simulink model "s_c107m32k_vlbi"  (R2018a)
settings: Solver=VariableStepDiscrete  StartTime=0.0  StopTime=(2^15)*10  RelTol=1e-3
undefined symbols (not defined in the file): fft_stages, n_bits_xengs
libraries: xbsIndex_r4 x23049, casper_library_misc x45, xps_library x4, casper_library_scopes x3, simulink x2
(part 24 of 201)

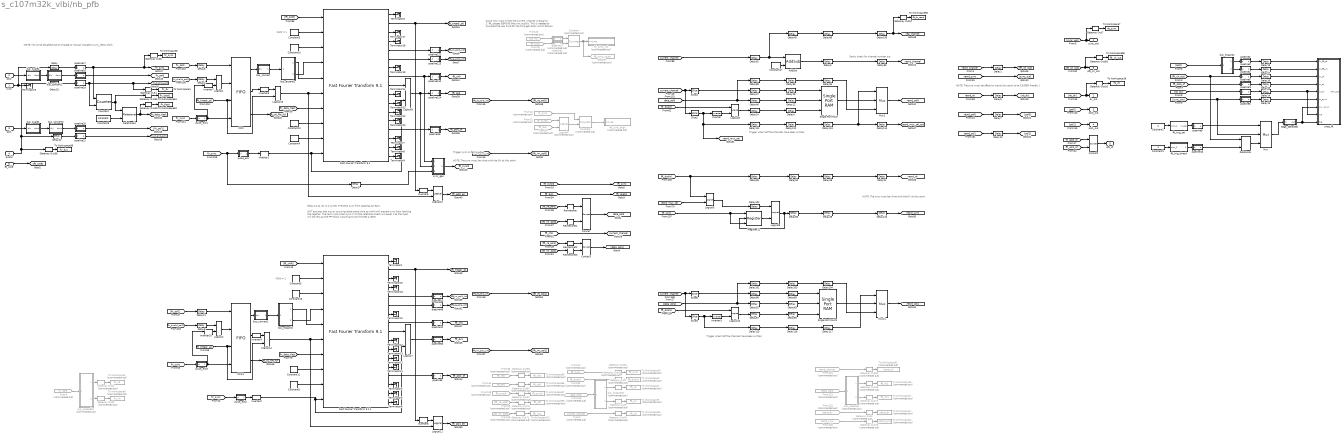
== system s_c107m32k_vlbi/nb_pfb ==
  note: FWD = 1
  note: NOTE: Init script Disabled due to change to manual change to sync_delay block
  note: NOTE: The sync must be inline with the DV at this point
  note: Trigger sync on falling edge
  note: NOT ensures that a sync occuring atthe same time as ch=0 will prevent
      | sync from latching the register. The next cycle when sync in =0 the relational check
      | will equal 1  as the input will be zero as the FFT block would have just finished a reset.
  note: Delay=2 as rst is 2 cycles. Prevents sync from popping out early
  note: Sanity check for channel number out
  note: Trigger when half the channels have been written
  note: Count how many times the current_channel
      | is equal to 2^fft_stages BEFORE the sync occurs.
      | This is needed to compute the new time for the time gen
      | block which follows.
  note: Trigger when half the channels have been written
  note: NOTE: The sync must be inline with the DV at this point
  note: FWD = 1
  note: NOTE: The sync must be offset by one at this point to be CASPER friendly :)
  sync : Inport
  pol0 : Inport  Port=2
  pol1 : Inport  Port=3
  dvalid : Inport  Port=4
  fft_shift : Inport  Port=5
  AddSub : xbsIndex_r4/AddSub  mode=Subtraction  use_carryin=off  use_carryout=off  en=off  latency=1  precision=User Defined  arith_type=Unsigned  n_bits=fft_stages-1  bin_pt=0  quantization=Truncate  overflow=Wrap  use_behavioral_HDL=off  hw_selection=Fabric  pipelined=off  dbl_ovrd=off  block_type=addsub
  Concat : xbsIndex_r4/Concat  num_inputs=2  dbl_ovrd=off  block_type=concat
  Concat2 : xbsIndex_r4/Concat  num_inputs=2  dbl_ovrd=off  block_type=concat
  Concat3 : xbsIndex_r4/Concat  num_inputs=2  dbl_ovrd=off  block_type=concat
  Constant1 : Constant  SampleTime=1
  Constant10 : xbsIndex_r4/Constant  const=1  gui_display_data_type=Boolean  arith_type=Boolean  n_bits=1  bin_pt=0  preci_type=Single  exp_width=8  frac_width=24  explicit_period=on  period=1  equ=P=C  opselect=C  inp2=PCIN>>17  opr=+  inp1=P  carry=CIN  dbl_ovrd=off  block_type=constant
  Constant11 : xbsIndex_r4/Constant  const=1  gui_display_data_type=Boolean  arith_type=Boolean  n_bits=18  bin_pt=17  preci_type=Single  exp_width=8  frac_width=24  explicit_period=on  period=1  equ=P=C  opselect=C  inp2=PCIN>>17  opr=+  inp1=P  carry=CIN  dbl_ovrd=off  block_type=constant
  Constant12 : xbsIndex_r4/Constant  const=1  gui_display_data_type=Boolean  arith_type=Boolean  n_bits=18  bin_pt=17  preci_type=Single  exp_width=8  frac_width=24  explicit_period=on  period=1  equ=P=C  opselect=C  inp2=PCIN>>17  opr=+  inp1=P  carry=CIN  dbl_ovrd=off  block_type=constant
  Constant13 : xbsIndex_r4/Constant  const=1  gui_display_data_type=Boolean  arith_type=Boolean  n_bits=1  bin_pt=0  preci_type=Single  exp_width=8  frac_width=24  explicit_period=on  period=1  equ=P=C  opselect=C  inp2=PCIN>>17  opr=+  inp1=P  carry=CIN  dbl_ovrd=off  block_type=constant
  Constant17 : xbsIndex_r4/Constant  const=2^(fft_stages-2)  gui_display_data_type=Fixed-point  arith_type=Unsigned  n_bits=fft_stages-1  bin_pt=0  preci_type=Single  exp_width=8  frac_width=24  explicit_period=on  period=1  equ=P=C  opselect=C  inp2=PCIN>>17  opr=+  inp1=P  carry=CIN  dbl_ovrd=off  block_type=constant
  Constant2 : Constant  SampleTime=1
  Constant3 : xbsIndex_r4/Constant  const=1  gui_display_data_type=Fixed-point  arith_type=Unsigned  n_bits=1  bin_pt=0  preci_type=Single  exp_width=8  frac_width=24  explicit_period=on  period=1  equ=P=C  opselect=C  inp2=PCIN>>17  opr=+  inp1=P  carry=CIN  dbl_ovrd=off  block_type=constant
  Constant4 : xbsIndex_r4/Constant  const=1.0  gui_display_data_type=Boolean  arith_type=Boolean  n_bits=16  bin_pt=14  preci_type=Single  exp_width=8  frac_width=24  explicit_period=on  period=1  equ=P=C  opselect=C  inp2=PCIN>>17  opr=+  inp1=P  carry=CIN  dbl_ovrd=off  block_type=constant
  Constant5 : xbsIndex_r4/Constant  const=1  gui_display_data_type=Fixed-point  arith_type=Unsigned  n_bits=1  bin_pt=0  preci_type=Single  exp_width=8  frac_width=24  explicit_period=on  period=1  equ=P=C  opselect=C  inp2=PCIN>>17  opr=+  inp1=P  carry=CIN  dbl_ovrd=off  block_type=constant
  Constant8 : xbsIndex_r4/Constant  const=1  gui_display_data_type=Boolean  arith_type=Boolean  n_bits=18  bin_pt=17  preci_type=Single  exp_width=8  frac_width=24  explicit_period=on  period=1  equ=P=C  opselect=C  inp2=PCIN>>17  opr=+  inp1=P  carry=CIN  dbl_ovrd=off  block_type=constant
  Constant9 : xbsIndex_r4/Constant  const=(2^(fft_stages-1))-1  gui_display_data_type=Fixed-point  arith_type=Unsigned  n_bits=fft_stages+1  bin_pt=0  preci_type=Single  exp_width=8  frac_width=24  explicit_period=on  period=1  equ=P=C  opselect=C  inp2=PCIN>>17  opr=+  inp1=P  carry=CIN  dbl_ovrd=off  block_type=constant
  Counter3 : xbsIndex_r4/Counter  cnt_type=Free Running  cnt_to=Inf  operation=Up  start_count=0  cnt_by_val=1  arith_type=Unsigned  n_bits=fft_stages-1  bin_pt=0  load_pin=off  rst=on  en=on  explicit_period=on  period=1  use_behavioral_HDL=off  implementation=Fabric  dbl_ovrd=off  block_type=counter
  Counter4 : xbsIndex_r4/Counter  Commented=on  cnt_type=Free Running  cnt_to=Inf  operation=Up  start_count=0  cnt_by_val=1  arith_type=Unsigned  n_bits=11  bin_pt=0  load_pin=off  rst=on  en=on  explicit_period=on  period=1  use_behavioral_HDL=off  implementation=DSP48  dbl_ovrd=off  block_type=counter
      settings: block_version=11.4
  Counter5 : xbsIndex_r4/Counter  Commented=on  cnt_type=Free Running  cnt_to=Inf  operation=Up  start_count=0  cnt_by_val=1  arith_type=Unsigned  n_bits=11  bin_pt=0  load_pin=off  rst=on  en=on  explicit_period=on  period=1  use_behavioral_HDL=off  implementation=DSP48  dbl_ovrd=off  block_type=counter
      settings: block_version=11.4
  Delay{,1,3..5,7,10,12..22,24,45..50,55,63,65,86..88,90..96,99..104,110..117} (52 alike) : xbsIndex_r4/Delay  rst=off  infoeditControl=Selection of Reset will increase slice count due to use of real FFs and instead of SRLs  en=off  latency=1  reg_retiming=off  dbl_ovrd=off  block_type=delay
      Delay1 settings: infoedit=Hardware notes: A delay line is a chain, each link of which is an SRL16 or SRL32 followed by a flip-flop.
      Delay10 settings: infoedit=Hardware notes: A delay line is a chain, each link of which is an SRL16 or SRL32 followed by a flip-flop.
      Delay100 settings: infoedit=Hardware notes: A delay line is a chain, each link of which is an SRL16 or SRL32 followed by a flip-flop.
      Delay101 settings: infoedit=Hardware notes: A delay line is a chain, each link of which is an SRL16 or SRL32 followed by a flip-flop.
      Delay102 settings: infoedit=Hardware notes: A delay line is a chain, each link of which is an SRL16 or SRL32 followed by a flip-flop.
      Delay103 settings: infoedit=Hardware notes: A delay line is a chain, each link of which is an SRL16 or SRL32 followed by a flip-flop.
      Delay104 settings: infoedit=Hardware notes: A delay line is a chain, each link of which is an SRL16 or SRL32 followed by a flip-flop.
      Delay110 settings: infoedit=Hardware notes: A delay line is a chain, each link of which is an SRL16 or SRL32 followed by a flip-flop.
      Delay111 settings: infoedit=Hardware notes: A delay line is a chain, each link of which is an SRL16 or SRL32 followed by a flip-flop.
      Delay112 settings: infoedit=Hardware notes: A delay line is a chain, each link of which is an SRL16 or SRL32 followed by a flip-flop.
      Delay113 settings: infoedit=Hardware notes: A delay line is a chain, each link of which is an SRL16 or SRL32 followed by a flip-flop.
      Delay114 settings: infoedit=Hardware notes: A delay line is a chain, each link of which is an SRL16 or SRL32 followed by a flip-flop.
      Delay115 settings: infoedit=Hardware notes: A delay line is a chain, each link of which is an SRL16 or SRL32 followed by a flip-flop.
      Delay116 settings: infoedit=Hardware notes: A delay line is a chain, each link of which is an SRL16 or SRL32 followed by a flip-flop.
      Delay117 settings: infoedit=Hardware notes: A delay line is a chain, each link of which is an SRL16 or SRL32 followed by a flip-flop.
      Delay12 settings: infoedit=Hardware notes: A delay line is a chain, each link of which is an SRL16 or SRL32 followed by a flip-flop.
      Delay13 settings: infoedit=Hardware notes: A delay line is a chain, each link of which is an SRL16 or SRL32 followed by a flip-flop.
      Delay14 settings: infoedit=Hardware notes: A delay line is a chain, each link of which is an SRL16 or SRL32 followed by a flip-flop.
      Delay15 settings: infoedit=Hardware notes: A delay line is a chain, each link of which is an SRL16 or SRL32 followed by a flip-flop.
      Delay16 settings: infoedit=Hardware notes: A delay line is a chain, each link of which is an SRL16 or SRL32 followed by a flip-flop.
      Delay17 settings: infoedit=Hardware notes: A delay line is a chain, each link of which is an SRL16 or SRL32 followed by a flip-flop.
      Delay18 settings: infoedit=Hardware notes: A delay line is a chain, each link of which is an SRL16 or SRL32 followed by a flip-flop.
      Delay19 settings: infoedit=Hardware notes: A delay line is a chain, each link of which is an SRL16 or SRL32 followed by a flip-flop.
      Delay21 settings: infoedit=Hardware notes: A delay line is a chain, each link of which is an SRL16 or SRL32 followed by a flip-flop.
      Delay24 settings: infoedit=Hardware notes: A delay line is a chain, each link of which is an SRL16 or SRL32 followed by a flip-flop.
      Delay3 settings: infoedit=Hardware notes: A delay line is a chain, each link of which is an SRL16 or SRL32 followed by a flip-flop.
      Delay4 settings: infoedit=Hardware notes: A delay line is a chain, each link of which is an SRL16 or SRL32 followed by a flip-flop.
      Delay45 settings: infoedit=Hardware notes: A delay line is a chain, each link of which is an SRL16 or SRL32 followed by a flip-flop.
      Delay46 settings: infoedit=Hardware notes: A delay line is a chain, each link of which is an SRL16 or SRL32 followed by a flip-flop.
      Delay47 settings: infoedit=Hardware notes: A delay line is a chain, each link of which is an SRL16 or SRL32 followed by a flip-flop.
      Delay48 settings: infoedit=Hardware notes: A delay line is a chain, each link of which is an SRL16 or SRL32 followed by a flip-flop.
      Delay49 settings: infoedit=Hardware notes: A delay line is a chain, each link of which is an SRL16 or SRL32 followed by a flip-flop.
      Delay5 settings: infoedit=Hardware notes: A delay line is a chain, each link of which is an SRL16 or SRL32 followed by a flip-flop.
      Delay50 settings: infoedit=Hardware notes: A delay line is a chain, each link of which is an SRL16 or SRL32 followed by a flip-flop.
      Delay55 settings: infoedit=Hardware notes: A delay line is a chain, each link of which is an SRL16 or SRL32 followed by a flip-flop.
      Delay63 settings: infoedit=Hardware notes: A delay line is a chain, each link of which is an SRL16 or SRL32 followed by a flip-flop.
      Delay65 settings: infoedit=Hardware notes: A delay line is a chain, each link of which is an SRL16 or SRL32 followed by a flip-flop.
      Delay7 settings: infoedit=Hardware notes: A delay line is a chain, each link of which is an SRL16 or SRL32 followed by a flip-flop.
      Delay86 settings: infoedit=Hardware notes: A delay line is a chain, each link of which is an SRL16 or SRL32 followed by a flip-flop.
      Delay87 settings: infoedit=Hardware notes: A delay line is a chain, each link of which is an SRL16 or SRL32 followed by a flip-flop.
      Delay88 settings: infoedit=Hardware notes: A delay line is a chain, each link of which is an SRL16 or SRL32 followed by a flip-flop.
      Delay90 settings: infoedit=Hardware notes: A delay line is a chain, each link of which is an SRL16 or SRL32 followed by a flip-flop.
      Delay91 settings: infoedit=Hardware notes: A delay line is a chain, each link of which is an SRL16 or SRL32 followed by a flip-flop.
      Delay92 settings: infoedit=Hardware notes: A delay line is a chain, each link of which is an SRL16 or SRL32 followed by a flip-flop.
      Delay93 settings: infoedit=Hardware notes: A delay line is a chain, each link of which is an SRL16 or SRL32 followed by a flip-flop.
      Delay94 settings: infoedit=Hardware notes: A delay line is a chain, each link of which is an SRL16 or SRL32 followed by a flip-flop.
      Delay95 settings: infoedit=Hardware notes: A delay line is a chain, each link of which is an SRL16 or SRL32 followed by a flip-flop.
      Delay96 settings: infoedit=Hardware notes: A delay line is a chain, each link of which is an SRL16 or SRL32 followed by a flip-flop.
      Delay99 settings: infoedit=Hardware notes: A delay line is a chain, each link of which is an SRL16 or SRL32 followed by a flip-flop.
  Delay{2,6,8,11} (4 alike) : xbsIndex_r4/Delay  rst=off  infoeditControl=Selection of Reset will increase slice count due to use of real FFs and instead of SRLs  en=off  latency=10  reg_retiming=off  dbl_ovrd=off  block_type=delay
      settings: infoedit=Hardware notes: A delay line is a chain, each link of which is an SRL16 or SRL32 followed by a flip-flop.
  Delay9 : xbsIndex_r4/Delay  rst=off  infoeditControl=Selection of Reset will increase slice count due to use of real FFs and instead of SRLs  en=off  latency=2  reg_retiming=off  dbl_ovrd=off  block_type=delay
      settings: infoedit=Hardware notes: A delay line is a chain, each link of which is an SRL16 or SRL32 followed by a flip-flop.
  FIFO : xbsIndex_r4/FIFO  mem_type=Distributed RAM  performance_options=First_Word_Fall_Through  embedded_registers=off  depth=16  percent_nbits=1  rst=on  rst_latency=1  en=off  use_dcount=off  use_percent_full_port=off  use_almost_empty=off  almost_empty_thresh=2  use_almost_full=off  use_rd_rst_busy=off  use_wr_rst_busy=off  almost_full_thresh=14  explicit_period=off  dbl_ovrd=off  block_type=fifo
  FIFO1 : xbsIndex_r4/FIFO  mem_type=Distributed RAM  performance_options=First_Word_Fall_Through  embedded_registers=off  depth=16  percent_nbits=1  rst=on  rst_latency=1  en=off  use_dcount=off  use_percent_full_port=off  use_almost_empty=off  almost_empty_thresh=2  use_almost_full=off  use_rd_rst_busy=off  use_wr_rst_busy=off  almost_full_thresh=14  explicit_period=off  dbl_ovrd=off  block_type=fifo
  "Fast Fourier Transform 9.1 " : xbsIndex_r4/Fast Fourier Transform 9.1   transform_length=32768  target_clock_frequency=240  target_data_throughput=50  implementation_options=pipelined_streaming_io  run_time_configurable_transform_length=off  phase_factor_width=18  scaling_options=scaled  rounding_modes=convergent_rounding  aclken=off  aresetn=on  output_ordering=natural_order  cyclic_prefix_insertion=off  throttle_scheme=nonrealtime  xk_index=on  ovflo=on  trim_axipin_name=on  memory_options_data=block_ram  memory_options_phase_factors=block_ram  number_of_stages_using_block_ram_for_data_and_phase_factors=6  memory_options_reorder=block_ram  memory_options_hybrid=off  complex_mult_type=use_mults_performance  butterfly_type=use_xtremedsp_slices  simulation_type=hybrid_sim  simulation_model=sysgen:xfftv9_cmodel  data_path_portlist={ 's_axis_data_tdata', 'm_axis_data_tdata', 'm_axis_status_tdata', 'event_fft_overflow' }  channels=1  input_ordering=natural_order  input_width=16  ip_name=Fast Fourier Transform  ip_version=9.1  dsptool_ready=true  ipcore_usecache=true  ipcore_useipmodelcache=true  wrapper_available=true  port_translation_map={ 'aclken' => 'en', 'aresetn' => 'rst'}  data_format=fixed_point  block_type=xfft_v9_1
  Fast Fourier Transform 9.1 1 : xbsIndex_r4/Fast Fourier Transform 9.1   transform_length=32768  target_clock_frequency=240  target_data_throughput=50  implementation_options=pipelined_streaming_io  run_time_configurable_transform_length=off  phase_factor_width=18  scaling_options=scaled  rounding_modes=convergent_rounding  aclken=off  aresetn=on  output_ordering=natural_order  cyclic_prefix_insertion=off  throttle_scheme=nonrealtime  xk_index=on  ovflo=on  trim_axipin_name=on  memory_options_data=block_ram  memory_options_phase_factors=block_ram  number_of_stages_using_block_ram_for_data_and_phase_factors=6  memory_options_reorder=block_ram  memory_options_hybrid=off  complex_mult_type=use_mults_performance  butterfly_type=use_xtremedsp_slices  simulation_type=hybrid_sim  simulation_model=sysgen:xfftv9_cmodel  data_path_portlist={ 's_axis_data_tdata', 'm_axis_data_tdata', 'm_axis_status_tdata', 'event_fft_overflow' }  channels=1  input_ordering=natural_order  input_width=16  ip_name=Fast Fourier Transform  ip_version=9.1  dsptool_ready=true  ipcore_usecache=true  ipcore_useipmodelcache=true  wrapper_available=true  port_translation_map={ 'aclken' => 'en', 'aresetn' => 'rst'}  data_format=fixed_point  block_type=xfft_v9_1
  From108 : From  Commented=on  GotoTag=fft_sync0  TagVisibility=global
  From123 : From  Commented=on  GotoTag=reord_pol0  TagVisibility=global
  From124 : From  Commented=on  GotoTag=reord_channel  TagVisibility=global
  From125 : From  Commented=on  GotoTag=reord_dv  TagVisibility=global
  From126 : From  Commented=on  GotoTag=reord_sync  TagVisibility=global
  From140 : From  Commented=on  GotoTag=data_pol0  TagVisibility=global
  From2 : From  Commented=on  GotoTag=current_channel  TagVisibility=global
  From20 : From  Commented=on  GotoTag=fft_sync  TagVisibility=global
  From26 : From  Commented=on  GotoTag=cnt_rst  TagVisibility=global
      settings: CloseFcn=tagdialog Close
  From28 : From  Commented=on  GotoTag=fft_re_pol0
  From30 : From  Commented=on  GotoTag=fft_dvalid  TagVisibility=global
  From31 : From  Commented=on  GotoTag=fft_sync0  TagVisibility=global
  From32 : From  Commented=on  GotoTag=fft_sync  TagVisibility=global
  From33 : From  Commented=on  GotoTag=fft_im_pol0
  From34 : From  Commented=on  GotoTag=fft_dv0  TagVisibility=global
  From38 : From  Commented=on  GotoTag=fft_ch0  TagVisibility=global
  From4 : From  Commented=on  GotoTag=fir_pol0  TagVisibility=global
  From40 : From  Commented=on  GotoTag=fft_dv0  TagVisibility=global
  From42 : From  Commented=on  GotoTag=fir_sync  TagVisibility=global
  Gateway Out{1,6..7,18,36,48,53,57,83} (9 alike) : xbsIndex_r4/Gateway Out  inherit_from_input=off  hdl_port=on  rows=1  columns=1  UseAsDAC=off  DACChannel='1'  interface=None  automatic_assignment=on  address_offset=hex2dec('00')  intf_name=''  intf_description=''  timing_constraint=None  locs_specified=off  LOCs={}  io_standard={}  block_type=gatewayout
  Gateway Out{2..5,8,15..17,34,37,50..52,66..67,70..71} (17 alike) : xbsIndex_r4/Gateway Out  Commented=on  inherit_from_input=off  hdl_port=on  rows=1  columns=1  UseAsDAC=off  DACChannel='1'  interface=None  automatic_assignment=on  address_offset=hex2dec('00')  intf_name=''  intf_description=''  timing_constraint=None  locs_specified=off  LOCs={}  io_standard={}  block_type=gatewayout
  Goto29 : Goto  Commented=on  GotoTag=fft_sync_count  TagVisibility=global
  Inverter{,1..3,5..10} (10 alike) : xbsIndex_r4/Inverter  en=off  latency=0  dbl_ovrd=off  block_type=inv
  Logical{1..2,5..14} (12 alike) : xbsIndex_r4/Logical  logical_function=AND  inputs=2  en=off  latency=0  precision=Full  arith_type=Unsigned  n_bits=16  bin_pt=0  align_bp=on  dbl_ovrd=off  block_type=logical
  Logical4 : xbsIndex_r4/Logical  Commented=on  logical_function=AND  inputs=2  en=off  latency=0  precision=Full  arith_type=Unsigned  n_bits=16  bin_pt=0  align_bp=on  dbl_ovrd=off  block_type=logical
  Mux : xbsIndex_r4/Mux  inputs=2  en=off  latency=1  precision=Full  arith_type=Unsigned  n_bits=16  bin_pt=14  quantization=Truncate  overflow=Wrap  dbl_ovrd=off  block_type=mux
  Mux1 : xbsIndex_r4/Mux  inputs=2  en=off  latency=1  precision=Full  arith_type=Unsigned  n_bits=16  bin_pt=14  quantization=Truncate  overflow=Wrap  dbl_ovrd=off  block_type=mux
  Mux11 : xbsIndex_r4/Mux  inputs=2  en=off  latency=1  precision=Full  arith_type=Unsigned  n_bits=16  bin_pt=14  quantization=Truncate  overflow=Wrap  dbl_ovrd=off  block_type=mux
  Register12 : xbsIndex_r4/Register  init=0  rst=on  en=on  dbl_ovrd=off  block_type=register
  Reinterpret{,1..3} (4 alike) : xbsIndex_r4/Reinterpret  force_arith_type=on  arith_type=Unsigned  force_bin_pt=on  bin_pt=0  block_type=reinterpret
  Relational : xbsIndex_r4/Relational  mode=a=b  op_type=Bool  en=off  latency=2  dbl_ovrd=off  block_type=relational
  Relational4 : xbsIndex_r4/Relational  mode=a=b  op_type=Bool  en=off  latency=1  dbl_ovrd=off  block_type=relational
  Single Port RAM : xbsIndex_r4/Single Port RAM  depth=2^(fft_stages-2)  initVector=0  distributed_mem=Block RAM  write_mode=Read Before Write  rst=off  init_reg=0  en=off  latency=1  optimize=Area  dbl_ovrd=off  block_type=spram
  Single Port RAM1 : xbsIndex_r4/Single Port RAM  depth=2^(fft_stages-2)  initVector=0  distributed_mem=Block RAM  write_mode=Read Before Write  rst=off  init_reg=0  en=off  latency=1  optimize=Area  dbl_ovrd=off  block_type=spram
  Slice2 : xbsIndex_r4/Slice  nbits=1  boolean_output=on  mode=Lower Bit Location + Width  bit1=0  base1=MSB of Input  bit0=fft_stages-2  base0=LSB of Input  dbl_ovrd=off  block_type=slice
  Slice3 : xbsIndex_r4/Slice  nbits=1  boolean_output=on  mode=Lower Bit Location + Width  bit1=0  base1=MSB of Input  bit0=fft_stages-2  base0=LSB of Input  dbl_ovrd=off  block_type=slice
  Slice4 : xbsIndex_r4/Slice  nbits=fft_stages-2  boolean_output=off  mode=Lower Bit Location + Width  bit1=0  base1=MSB of Input  bit0=0  base0=LSB of Input  dbl_ovrd=off  block_type=slice
  Slice6 : xbsIndex_r4/Slice  nbits=fft_stages-2  boolean_output=off  mode=Lower Bit Location + Width  bit1=0  base1=MSB of Input  bit0=0  base0=LSB of Input  dbl_ovrd=off  block_type=slice
  Terminator{1..13,15..24} (23 alike) : Terminator
  To Workspace1 : ToWorkspace  VariableName=fir_dv  SaveFormat=Timeseries  SampleTime=-1
  To Workspace15 : ToWorkspace  Commented=on  VariableName=fft_re1  SaveFormat=Timeseries  SampleTime=-1
  To Workspace16 : ToWorkspace  Commented=on  VariableName=fft_sync  SaveFormat=Timeseries  SampleTime=-1
  To Workspace17 : ToWorkspace  Commented=on  VariableName=fft_im1  SaveFormat=Timeseries  SampleTime=-1
  To Workspace19 : ToWorkspace  VariableName=nb_dv  SaveFormat=Timeseries  SampleTime=-1
  To Workspace2 : ToWorkspace  Commented=on  VariableName=fft_re  SaveFormat=Timeseries  SampleTime=-1
  To Workspace3 : ToWorkspace  Commented=on  VariableName=fft_dvalid  SaveFormat=Timeseries  SampleTime=-1
  To Workspace32 : ToWorkspace  Commented=on  VariableName=fft_ch  SaveFormat=Timeseries  SampleTime=-1
  To Workspace36 : ToWorkspace  VariableName=fir_dv1  SaveFormat=Timeseries  SampleTime=-1
  To Workspace37 : ToWorkspace  Commented=on  VariableName=fft_sync0  SaveFormat=Timeseries  SampleTime=-1
  To Workspace4 : ToWorkspace  Commented=on  VariableName=fir_re  SaveFormat=Timeseries  SampleTime=-1
  To Workspace42 : ToWorkspace  Commented=on  VariableName=reord_sync  SaveFormat=Timeseries  SampleTime=-1
  To Workspace47 : ToWorkspace  Commented=on  VariableName=reord_dv  SaveFormat=Timeseries  SampleTime=-1
  To Workspace5 : ToWorkspace  Commented=on  VariableName=fft_im  SaveFormat=Timeseries  SampleTime=-1
  To Workspace51 : ToWorkspace  Commented=on  VariableName=reord_ch  SaveFormat=Timeseries  SampleTime=-1
  To Workspace53 : ToWorkspace  VariableName=fir_tlast  SaveFormat=Timeseries  SampleTime=-1
  To Workspace54 : ToWorkspace  VariableName=fir_tlast1  SaveFormat=Timeseries  SampleTime=-1
  To Workspace58 : ToWorkspace  VariableName=fft_ch_reord  SaveFormat=Timeseries  SampleTime=-1
  To Workspace6 : ToWorkspace  VariableName=fir_sync  SaveFormat=Timeseries  SampleTime=-1
  To Workspace65 : ToWorkspace  Commented=on  VariableName=fft_ch0  SaveFormat=Timeseries  SampleTime=-1
  To Workspace66 : ToWorkspace  Commented=on  VariableName=fft_dv0  SaveFormat=Timeseries  SampleTime=-1
  To Workspace69 : ToWorkspace  Commented=on  VariableName=fft_re2  SaveFormat=Timeseries  SampleTime=-1
  To Workspace7 : ToWorkspace  VariableName=nb_sync  SaveFormat=Timeseries  SampleTime=-1
  To Workspace70 : ToWorkspace  Commented=on  VariableName=fft_im2  SaveFormat=Timeseries  SampleTime=-1
  To Workspace8 : ToWorkspace  Commented=on  VariableName=fir_im  SaveFormat=Timeseries  SampleTime=-1
  To Workspace85 : ToWorkspace  VariableName=fft_ch_out  SaveFormat=Timeseries  SampleTime=-1
  bus_convert : Subsystem  AncestorBlock=casper_library_bus/bus_convert  mask(bus_convert){n_bits_in=[18 18], bin_pt_in=[17 17], cmplx=off, n_bits_out=[22 22], bin_pt_out=[21 21], quantization=0, overflow=0, csp_latency=0, of=off, misc=off}
      mask prompts: n_bits_in "input bit widths"; bin_pt_in "input binary points"; cmplx "input complex"; n_bits_out "output bit widths"; bin_pt_out "output binary points"; quantization "quantization strategy (Truncate=0, Round  (unbiased: +/- Inf)=1, Round (unbiased: Even Values)=2)"; overflow "overflow strategy (Wrap=0, Saturate=1, Flag as error=2)"; csp_latency "latency"; of "overflow indication"; misc "misc support"
      mask help: Convert components of busses
      mask init: same as s_c107m32k_vlbi/DDC/bus_convert
  bus_convert1 : Subsystem  AncestorBlock=casper_library_bus/bus_convert  mask(bus_convert){n_bits_in=[18 18], bin_pt_in=[17 17], cmplx=off, n_bits_out=[22 22], bin_pt_out=[21 21], quantization=0, overflow=0, csp_latency=0, of=off, misc=off}
      mask prompts: n_bits_in "input bit widths"; bin_pt_in "input binary points"; cmplx "input complex"; n_bits_out "output bit widths"; bin_pt_out "output binary points"; quantization "quantization strategy (Truncate=0, Round  (unbiased: +/- Inf)=1, Round (unbiased: Even Values)=2)"; overflow "overflow strategy (Wrap=0, Saturate=1, Flag as error=2)"; csp_latency "latency"; of "overflow indication"; misc "misc support"
      mask help: Convert components of busses
      mask init: same as s_c107m32k_vlbi/DDC/bus_convert
  bus_convert2 : Subsystem  AncestorBlock=casper_library_bus/bus_convert  mask(bus_convert){n_bits_in=[18], bin_pt_in=18, cmplx=on, n_bits_out=18, bin_pt_out=17, quantization=2, overflow=1, csp_latency=1, of=off, misc=off}
      mask prompts: n_bits_in "input bit widths"; bin_pt_in "input binary points"; cmplx "input complex"; n_bits_out "output bit widths"; bin_pt_out "output binary points"; quantization "quantization strategy (Truncate=0, Round  (unbiased: +/- Inf)=1, Round (unbiased: Even Values)=2)"; overflow "overflow strategy (Wrap=0, Saturate=1, Flag as error=2)"; csp_latency "latency"; of "overflow indication"; misc "misc support"
      mask help: Convert components of busses
      mask init: same as s_c107m32k_vlbi/DDC/bus_convert
  bus_convert3 : Subsystem  AncestorBlock=casper_library_bus/bus_convert  mask(bus_convert){n_bits_in=[18], bin_pt_in=18, cmplx=on, n_bits_out=18, bin_pt_out=17, quantization=2, overflow=1, csp_latency=1, of=off, misc=off}
      mask prompts: n_bits_in "input bit widths"; bin_pt_in "input binary points"; cmplx "input complex"; n_bits_out "output bit widths"; bin_pt_out "output binary points"; quantization "quantization strategy (Truncate=0, Round  (unbiased: +/- Inf)=1, Round (unbiased: Even Values)=2)"; overflow "overflow strategy (Wrap=0, Saturate=1, Flag as error=2)"; csp_latency "latency"; of "overflow indication"; misc "misc support"
      mask help: Convert components of busses
      mask init: same as s_c107m32k_vlbi/DDC/bus_convert
  bus_expand1 : Subsystem  mask(bus_expand){mode=divisions of equal size, outputNum=2, outputWidth=22, outputBinaryPt=21, outputArithmeticType=1, show_format=off, outputToWorkspace=off, variablePrefix=out, outputToModelAsWell=on}
      mask prompts: outputNum "Number of outputs:"; outputWidth "Output width:"; outputBinaryPt "Output binary point position:"; outputArithmeticType "Output arithmetic type (ufix=0, fix=1, bool=2):"; show_format "Print format string?"; outputToWorkspace "Output to workspace?"; variablePrefix "Variable name prefix:"; outputToModelAsWell "Output to model as well?"
      mask help:
      | Expands a 'bus' made using a bus_create or Xilinx
      | concat block.
      | The input will be divided into the specified number
      | of outputs with the specified arithmetic types.
      | Divisions are made from most significant bit.
      mask init: same as s_c107m32k_vlbi/bus_expand1
      settings: AttributesFormatString=2 outputs
      mask TypeOptions mode: divisions of equal size | divisions of arbitrary size
      mask Callback mode: bus_expand_callback();
      mask Callback outputWidth: bus_expand_callback();
      mask Callback outputToWorkspace: bus_expand_callback();
  bus_expand13 : Subsystem  Commented=on  mask(bus_expand){mode=divisions of equal size, outputNum=2, outputWidth=18, outputBinaryPt=17, outputArithmeticType=1, show_format=off, outputToWorkspace=off, variablePrefix=out, outputToModelAsWell=on}
      mask prompts: outputNum "Number of outputs:"; outputWidth "Output width:"; outputBinaryPt "Output binary point position:"; outputArithmeticType "Output arithmetic type (ufix=0, fix=1, bool=2):"; show_format "Print format string?"; outputToWorkspace "Output to workspace?"; variablePrefix "Variable name prefix:"; outputToModelAsWell "Output to model as well?"
      mask help:
      | Expands a 'bus' made using a bus_create or Xilinx
      | concat block.
      | The input will be divided into the specified number
      | of outputs with the specified arithmetic types.
      | Divisions are made from most significant bit.
      mask init: same as s_c107m32k_vlbi/bus_expand1
      settings: AttributesFormatString=2 outputs
      mask TypeOptions mode: divisions of equal size | divisions of arbitrary size
      mask Callback mode: bus_expand_callback();
      mask Callback outputWidth: bus_expand_callback();
      mask Callback outputToWorkspace: bus_expand_callback();
  bus_expand16 : Subsystem  Commented=on  mask(bus_expand){mode=divisions of equal size, outputNum=2, outputWidth=18, outputBinaryPt=17, outputArithmeticType=1, show_format=off, outputToWorkspace=off, variablePrefix=out, outputToModelAsWell=on}
      mask prompts: outputNum "Number of outputs:"; outputWidth "Output width:"; outputBinaryPt "Output binary point position:"; outputArithmeticType "Output arithmetic type (ufix=0, fix=1, bool=2):"; show_format "Print format string?"; outputToWorkspace "Output to workspace?"; variablePrefix "Variable name prefix:"; outputToModelAsWell "Output to model as well?"
      mask help:
      | Expands a 'bus' made using a bus_create or Xilinx
      | concat block.
      | The input will be divided into the specified number
      | of outputs with the specified arithmetic types.
      | Divisions are made from most significant bit.
      mask init: same as s_c107m32k_vlbi/bus_expand1
      settings: AttributesFormatString=2 outputs
      mask TypeOptions mode: divisions of equal size | divisions of arbitrary size
      mask Callback mode: bus_expand_callback();
      mask Callback outputWidth: bus_expand_callback();
      mask Callback outputToWorkspace: bus_expand_callback();
  bus_expand2 : Subsystem  mask(bus_expand){mode=divisions of equal size, outputNum=2, outputWidth=22, outputBinaryPt=21, outputArithmeticType=1, show_format=off, outputToWorkspace=off, variablePrefix=out, outputToModelAsWell=on}
      mask prompts: outputNum "Number of outputs:"; outputWidth "Output width:"; outputBinaryPt "Output binary point position:"; outputArithmeticType "Output arithmetic type (ufix=0, fix=1, bool=2):"; show_format "Print format string?"; outputToWorkspace "Output to workspace?"; variablePrefix "Variable name prefix:"; outputToModelAsWell "Output to model as well?"
      mask help:
      | Expands a 'bus' made using a bus_create or Xilinx
      | concat block.
      | The input will be divided into the specified number
      | of outputs with the specified arithmetic types.
      | Divisions are made from most significant bit.
      mask init: same as s_c107m32k_vlbi/bus_expand1
      settings: AttributesFormatString=2 outputs
      mask TypeOptions mode: divisions of equal size | divisions of arbitrary size
      mask Callback mode: bus_expand_callback();
      mask Callback outputWidth: bus_expand_callback();
      mask Callback outputToWorkspace: bus_expand_callback();
  bus_expand3 : Subsystem  Commented=on  mask(bus_expand){mode=divisions of equal size, outputNum=2, outputWidth=18, outputBinaryPt=17, outputArithmeticType=1, show_format=off, outputToWorkspace=off, variablePrefix=out, outputToModelAsWell=on}
      mask prompts: outputNum "Number of outputs:"; outputWidth "Output width:"; outputBinaryPt "Output binary point position:"; outputArithmeticType "Output arithmetic type (ufix=0, fix=1, bool=2):"; show_format "Print format string?"; outputToWorkspace "Output to workspace?"; variablePrefix "Variable name prefix:"; outputToModelAsWell "Output to model as well?"
      mask help:
      | Expands a 'bus' made using a bus_create or Xilinx
      | concat block.
      | The input will be divided into the specified number
      | of outputs with the specified arithmetic types.
      | Divisions are made from most significant bit.
      mask init: same as s_c107m32k_vlbi/bus_expand1
      settings: AttributesFormatString=2 outputs
      mask TypeOptions mode: divisions of equal size | divisions of arbitrary size
      mask Callback mode: bus_expand_callback();
      mask Callback outputWidth: bus_expand_callback();
      mask Callback outputToWorkspace: bus_expand_callback();
  bus_expand4 : Subsystem  mask(bus_expand){mode=divisions of equal size, outputNum=2, outputWidth=22, outputBinaryPt=21, outputArithmeticType=1, show_format=off, outputToWorkspace=off, variablePrefix=out, outputToModelAsWell=on}
      mask prompts: outputNum "Number of outputs:"; outputWidth "Output width:"; outputBinaryPt "Output binary point position:"; outputArithmeticType "Output arithmetic type (ufix=0, fix=1, bool=2):"; show_format "Print format string?"; outputToWorkspace "Output to workspace?"; variablePrefix "Variable name prefix:"; outputToModelAsWell "Output to model as well?"
      mask help:
      | Expands a 'bus' made using a bus_create or Xilinx
      | concat block.
      | The input will be divided into the specified number
      | of outputs with the specified arithmetic types.
      | Divisions are made from most significant bit.
      mask init: same as s_c107m32k_vlbi/bus_expand1
      settings: AttributesFormatString=2 outputs
      mask TypeOptions mode: divisions of equal size | divisions of arbitrary size
      mask Callback mode: bus_expand_callback();
      mask Callback outputWidth: bus_expand_callback();
      mask Callback outputToWorkspace: bus_expand_callback();
  bus_scale1 : Subsystem  AncestorBlock=casper_library_bus/bus_scale  mask(bus_scale){n_bits_in=[18], bin_pt_in=17, type_in=1, cmplx=on, scale_factor=-1, misc=off}
      mask prompts: n_bits_in "input bit widths"; bin_pt_in "input binary points"; type_in "input types"; cmplx "input complex"; scale_factor "scale factor (2^?)"; misc "misc support"
      mask help: Convert components of busses
      mask init:
      | bus_scale_init(gcb, ...
      |     'n_bits_in', n_bits_in, ...
      |     'bin_pt_in', bin_pt_in, ...
      |     'type_in', type_in, ...
      |     'cmplx', cmplx, ...
      |     'scale_factor', scale_factor, ...
      |     'misc', misc);
  bus_scale2 : Subsystem  AncestorBlock=casper_library_bus/bus_scale  mask(bus_scale){n_bits_in=[18], bin_pt_in=17, type_in=1, cmplx=on, scale_factor=-1, misc=off}
      mask prompts: n_bits_in "input bit widths"; bin_pt_in "input binary points"; type_in "input types"; cmplx "input complex"; scale_factor "scale factor (2^?)"; misc "misc support"
      mask help: Convert components of busses
      mask init:
      | bus_scale_init(gcb, ...
      |     'n_bits_in', n_bits_in, ...
      |     'bin_pt_in', bin_pt_in, ...
      |     'type_in', type_in, ...
      |     'cmplx', cmplx, ...
      |     'scale_factor', scale_factor, ...
      |     'misc', misc);
  edge_detect65 : Subsystem  mask(edge_detect){edge=Rising, polarity=Active High, x_in=[0 0.08 0.08 0.16 0.16 0.24 0.24 0.32 0.32 0.4], y_in=[-1 -1  1  1  1  1  1  1  1  1], x_out=[0.6 0.68 0.68 0.76 0.76 0.84 0.84 0.92 0.92 1], y_out=[-1 -1  1  1 -1 -1 -1 -1 -1 -1]}
      mask prompts: edge "Edge Type"; polarity "Output Polarity"; x_in "Input X Positions"; y_in "Input Y Positions"; x_out "Output X Positions"; y_out "Output Y Positions"
      mask help: Output is active for one-cycle after each edge of the specified type (i.e. rising, falling or both).
      mask init: same as s_c107m32k_vlbi/edge_detect1
      settings: AttributesFormatString=|
      | rising edges
      | active high
      mask Help: Output is active for one-cycle after each edge of the specified type (i.e. rising, falling, or both).  Latency is zero.
      mask TypeOptions edge: Rising | Falling | Both
      mask TypeOptions polarity: Active High | Active Low
      mask Display:
      | plot(x_in_num,0.5+y_in_num*0.2);
      | plot(x_out_num,0.5+y_out_num*0.2);
  fft_sync_align : Subsystem  Tag=xps:sw_reg  Commented=on  AncestorBlock=xps_library/Memory/software_register  mask(swreg){io_dir=To Processor, io_delay=0, init_val=0, sample_period=1, names=reg, bitwidths=11, bin_pts=0, arith_types=0, sim_port=off, show_format=on}
      mask prompts: io_dir "I/O direction"; io_delay "I/O delay"; init_val "Initial Value"; sample_period "Sample period"; names "Bitfield names [msb...lsb]"; bitwidths "Bitfield widths"; bin_pts "Bitfield binary pts"; arith_types "Bitfield types, ufix=0, fix=1, bool=2"; sim_port "Provide sim input/output?"; show_format "Print format string?"
      mask help: A 32-bit software-accessible register. Can be divided into bitfields of varying widths and types using the fields in the block mask.
      mask init:
      | swreg_init(gcb)
      settings: AttributesFormatString=1output:uf11.0 = 11 bits
      mask TypeOptions io_dir: To Processor | From Processor
      mask Callback io_dir:
      | mask_enables = get_param(gcb, 'MaskEnables');
      | mask_names = get_param(gcb, 'MaskNames');
      | if strcmp(get_param(gcb, 'io_dir'), 'To Processor'),
      |     mask_enables{ismember(mask_names, 'sample_period')} = 'off';
      | else
      |     mask_enables{ismember(mask_names, 'sample_period')} = 'on';
      | end
      | set_param(gcb, 'MaskEnables', mask_enables);
      mask DialogControl ParameterTabVar0 Prompt: Setup
  fft_sync_cnt : Subsystem  Tag=xps:sw_reg  Commented=on  AncestorBlock=xps_library/Memory/software_register  mask(swreg){io_dir=To Processor, io_delay=0, init_val=0, sample_period=1, names=reg, bitwidths=11, bin_pts=0, arith_types=0, sim_port=off, show_format=on}
      mask prompts: io_dir "I/O direction"; io_delay "I/O delay"; init_val "Initial Value"; sample_period "Sample period"; names "Bitfield names [msb...lsb]"; bitwidths "Bitfield widths"; bin_pts "Bitfield binary pts"; arith_types "Bitfield types, ufix=0, fix=1, bool=2"; sim_port "Provide sim input/output?"; show_format "Print format string?"
      mask help: A 32-bit software-accessible register. Can be divided into bitfields of varying widths and types using the fields in the block mask.
      mask init:
      | swreg_init(gcb)
      settings: AttributesFormatString=1output:uf11.0 = 11 bits
      mask TypeOptions io_dir: To Processor | From Processor
      mask Callback io_dir:
      | mask_enables = get_param(gcb, 'MaskEnables');
      | mask_names = get_param(gcb, 'MaskNames');
      | if strcmp(get_param(gcb, 'io_dir'), 'To Processor'),
      |     mask_enables{ismember(mask_names, 'sample_period')} = 'off';
      | else
      |     mask_enables{ismember(mask_names, 'sample_period')} = 'on';
      | end
      | set_param(gcb, 'MaskEnables', mask_enables);
      mask DialogControl ParameterTabVar0 Prompt: Setup
  fft_trig_sel : Subsystem  Tag=xps:sw_reg  AncestorBlock=xps_library/Memory/software_register  mask(swreg){io_dir=From Processor, io_delay=0, init_val=0, sample_period=1, names=[sel], bitwidths=[1], bin_pts=0, arith_types=2, sim_port=on, show_format=on}
      mask prompts: io_dir "I/O direction"; io_delay "I/O delay"; init_val "Initial Value"; sample_period "Sample period"; names "Bitfield names [msb...lsb]"; bitwidths "Bitfield widths"; bin_pts "Bitfield binary pts"; arith_types "Bitfield types, ufix=0, fix=1, bool=2"; sim_port "Provide sim input/output?"; show_format "Print format string?"
      mask help: A 32-bit software-accessible register. Can be divided into bitfields of varying widths and types using the fields in the block mask.
      mask init:
      | swreg_init(gcb)
      settings: AttributesFormatString=1input:b = 1 bits
      mask TypeOptions io_dir: To Processor | From Processor
      mask Callback io_dir:
      | mask_enables = get_param(gcb, 'MaskEnables');
      | mask_names = get_param(gcb, 'MaskNames');
      | if strcmp(get_param(gcb, 'io_dir'), 'To Processor'),
      |     mask_enables{ismember(mask_names, 'sample_period')} = 'off';
      | else
      |     mask_enables{ismember(mask_names, 'sample_period')} = 'on';
      | end
      | set_param(gcb, 'MaskEnables', mask_enables);
      mask DialogControl ParameterTabVar0 Prompt: Setup
  fft_trig_thresh : Subsystem  Tag=xps:sw_reg  AncestorBlock=xps_library/Memory/software_register  mask(swreg){io_dir=From Processor, io_delay=0, init_val=0, sample_period=1, names=[threshold], bitwidths=[15], bin_pts=0, arith_types=0, sim_port=on, show_format=on}
      mask prompts: io_dir "I/O direction"; io_delay "I/O delay"; init_val "Initial Value"; sample_period "Sample period"; names "Bitfield names [msb...lsb]"; bitwidths "Bitfield widths"; bin_pts "Bitfield binary pts"; arith_types "Bitfield types, ufix=0, fix=1, bool=2"; sim_port "Provide sim input/output?"; show_format "Print format string?"
      mask help: A 32-bit software-accessible register. Can be divided into bitfields of varying widths and types using the fields in the block mask.
      mask init:
      | swreg_init(gcb)
      settings: AttributesFormatString=1input:uf15.0 = 15 bits
      mask TypeOptions io_dir: To Processor | From Processor
      mask Callback io_dir:
      | mask_enables = get_param(gcb, 'MaskEnables');
      | mask_names = get_param(gcb, 'MaskNames');
      | if strcmp(get_param(gcb, 'io_dir'), 'To Processor'),
      |     mask_enables{ismember(mask_names, 'sample_period')} = 'off';
      | else
      |     mask_enables{ismember(mask_names, 'sample_period')} = 'on';
      | end
      | set_param(gcb, 'MaskEnables', mask_enables);
      mask DialogControl ParameterTabVar0 Prompt: Setup
  pipeline1 : Subsystem  Commented=on  AncestorBlock=casper_library_delays/pipeline  mask(pipeline){latency=2}
      mask help:
      | An explicitly laid-out delay line to avoid mapping to SRL16s
      | for use in pipelining to help achieve timing closure.
      mask init:
      | pipeline_init(gcb,'latency',latency);
      settings: AttributesFormatString=Latency = %<latency>
      mask Display:
      | port_label('input', 1, 'd');
      | port_label('output', 1, 'q');
      | disp(['Z^-', num2str(latency)]);
  pipeline10 : Subsystem  Tag=cmac_delinked  mask(pipeline){csp_latency=2}
      mask prompts: csp_latency "Latency"
      mask help:
      | An explicitly laid-out delay line to avoid mapping to SRL16s
      | for use in pipelining to help achieve timing closure.
      mask init:
      | pipeline_init(gcb,'latency',csp_latency);
      settings: AttributesFormatString=Latency = %<latency>
      mask Display:
      | port_label('input', 1, 'd');
      | port_label('output', 1, 'q');
      | disp(['Z^-', num2str(csp_latency)]);
  pipeline110 : Subsystem  Tag=cmac_delinked  mask(pipeline){csp_latency=2}
      mask prompts: csp_latency "Latency"
      mask help:
      | An explicitly laid-out delay line to avoid mapping to SRL16s
      | for use in pipelining to help achieve timing closure.
      mask init:
      | pipeline_init(gcb,'latency',csp_latency);
      settings: AttributesFormatString=Latency = %<latency>
      mask Display:
      | port_label('input', 1, 'd');
      | port_label('output', 1, 'q');
      | disp(['Z^-', num2str(csp_latency)]);
  pipeline12 : Subsystem  Tag=cmac_delinked  mask(pipeline){csp_latency=2}
      mask prompts: csp_latency "Latency"
      mask help:
      | An explicitly laid-out delay line to avoid mapping to SRL16s
      | for use in pipelining to help achieve timing closure.
      mask init:
      | pipeline_init(gcb,'latency',csp_latency);
      settings: AttributesFormatString=Latency = %<latency>
      mask Display:
      | port_label('input', 1, 'd');
      | port_label('output', 1, 'q');
      | disp(['Z^-', num2str(csp_latency)]);
  pipeline122 : Subsystem  Tag=cmac_delinked  mask(pipeline){csp_latency=2}
      mask prompts: csp_latency "Latency"
      mask help:
      | An explicitly laid-out delay line to avoid mapping to SRL16s
      | for use in pipelining to help achieve timing closure.
      mask init:
      | pipeline_init(gcb,'latency',csp_latency);
      settings: AttributesFormatString=Latency = %<latency>
      mask Display:
      | port_label('input', 1, 'd');
      | port_label('output', 1, 'q');
      | disp(['Z^-', num2str(csp_latency)]);
  pipeline123 : Subsystem  Tag=cmac_delinked  mask(pipeline){csp_latency=2}
      mask prompts: csp_latency "Latency"
      mask help:
      | An explicitly laid-out delay line to avoid mapping to SRL16s
      | for use in pipelining to help achieve timing closure.
      mask init:
      | pipeline_init(gcb,'latency',csp_latency);
      settings: AttributesFormatString=Latency = %<latency>
      mask Display:
      | port_label('input', 1, 'd');
      | port_label('output', 1, 'q');
      | disp(['Z^-', num2str(csp_latency)]);
  pipeline124 : Subsystem  Tag=cmac_delinked  mask(pipeline){csp_latency=2}
      mask prompts: csp_latency "Latency"
      mask help:
      | An explicitly laid-out delay line to avoid mapping to SRL16s
      | for use in pipelining to help achieve timing closure.
      mask init:
      | pipeline_init(gcb,'latency',csp_latency);
      settings: AttributesFormatString=Latency = %<latency>
      mask Display:
      | port_label('input', 1, 'd');
      | port_label('output', 1, 'q');
      | disp(['Z^-', num2str(csp_latency)]);
  pipeline16 : Subsystem  Tag=cmac_delinked  mask(pipeline){csp_latency=2}
      mask prompts: csp_latency "Latency"
      mask help:
      | An explicitly laid-out delay line to avoid mapping to SRL16s
      | for use in pipelining to help achieve timing closure.
      mask init:
      | pipeline_init(gcb,'latency',csp_latency);
      settings: AttributesFormatString=Latency = %<latency>
      mask Display:
      | port_label('input', 1, 'd');
      | port_label('output', 1, 'q');
      | disp(['Z^-', num2str(csp_latency)]);
  pipeline17 : Subsystem  Tag=cmac_delinked  mask(pipeline){csp_latency=2}
      mask prompts: csp_latency "Latency"
      mask help:
      | An explicitly laid-out delay line to avoid mapping to SRL16s
      | for use in pipelining to help achieve timing closure.
      mask init:
      | pipeline_init(gcb,'latency',csp_latency);
      settings: AttributesFormatString=Latency = %<latency>
      mask Display:
      | port_label('input', 1, 'd');
      | port_label('output', 1, 'q');
      | disp(['Z^-', num2str(csp_latency)]);
  pipeline18 : Subsystem  Tag=cmac_delinked  mask(pipeline){csp_latency=2}
      mask prompts: csp_latency "Latency"
      mask help:
      | An explicitly laid-out delay line to avoid mapping to SRL16s
      | for use in pipelining to help achieve timing closure.
      mask init:
      | pipeline_init(gcb,'latency',csp_latency);
      settings: AttributesFormatString=Latency = %<latency>
      mask Display:
      | port_label('input', 1, 'd');
      | port_label('output', 1, 'q');
      | disp(['Z^-', num2str(csp_latency)]);
  pipeline19 : Subsystem  Tag=cmac_delinked  mask(pipeline){csp_latency=2}
      mask prompts: csp_latency "Latency"
      mask help:
      | An explicitly laid-out delay line to avoid mapping to SRL16s
      | for use in pipelining to help achieve timing closure.
      mask init:
      | pipeline_init(gcb,'latency',csp_latency);
      settings: AttributesFormatString=Latency = %<latency>
      mask Display:
      | port_label('input', 1, 'd');
      | port_label('output', 1, 'q');
      | disp(['Z^-', num2str(csp_latency)]);
  pipeline2 : Subsystem  Tag=cmac_delinked  mask(pipeline){csp_latency=2}
      mask prompts: csp_latency "Latency"
      mask help:
      | An explicitly laid-out delay line to avoid mapping to SRL16s
      | for use in pipelining to help achieve timing closure.
      mask init:
      | pipeline_init(gcb,'latency',csp_latency);
      settings: AttributesFormatString=Latency = %<latency>
      mask Display:
      | port_label('input', 1, 'd');
      | port_label('output', 1, 'q');
      | disp(['Z^-', num2str(csp_latency)]);
  pipeline20 : Subsystem  Tag=cmac_delinked  mask(pipeline){csp_latency=2}
      mask prompts: csp_latency "Latency"
      mask help:
      | An explicitly laid-out delay line to avoid mapping to SRL16s
      | for use in pipelining to help achieve timing closure.
      mask init:
      | pipeline_init(gcb,'latency',csp_latency);
      settings: AttributesFormatString=Latency = %<latency>
      mask Display:
      | port_label('input', 1, 'd');
      | port_label('output', 1, 'q');
      | disp(['Z^-', num2str(csp_latency)]);
  pipeline21 : Subsystem  Tag=cmac_delinked  mask(pipeline){csp_latency=2}
      mask prompts: csp_latency "Latency"
      mask help:
      | An explicitly laid-out delay line to avoid mapping to SRL16s
      | for use in pipelining to help achieve timing closure.
      mask init:
      | pipeline_init(gcb,'latency',csp_latency);
      settings: AttributesFormatString=Latency = %<latency>
      mask Display:
      | port_label('input', 1, 'd');
      | port_label('output', 1, 'q');
      | disp(['Z^-', num2str(csp_latency)]);
  pipeline27 : Subsystem  Commented=on  AncestorBlock=casper_library_delays/pipeline  mask(pipeline){latency=2}
      mask help:
      | An explicitly laid-out delay line to avoid mapping to SRL16s
      | for use in pipelining to help achieve timing closure.
      mask init:
      | pipeline_init(gcb,'latency',latency);
      settings: AttributesFormatString=Latency = %<latency>
      mask Display:
      | port_label('input', 1, 'd');
      | port_label('output', 1, 'q');
      | disp(['Z^-', num2str(latency)]);
  pipeline3 : Subsystem  Tag=cmac_delinked  mask(pipeline){csp_latency=2}
      mask prompts: csp_latency "Latency"
      mask help:
      | An explicitly laid-out delay line to avoid mapping to SRL16s
      | for use in pipelining to help achieve timing closure.
      mask init:
      | pipeline_init(gcb,'latency',csp_latency);
      settings: AttributesFormatString=Latency = %<latency>
      mask Display:
      | port_label('input', 1, 'd');
      | port_label('output', 1, 'q');
      | disp(['Z^-', num2str(csp_latency)]);
  pipeline4 : Subsystem  Tag=cmac_delinked  mask(pipeline){csp_latency=2}
      mask prompts: csp_latency "Latency"
      mask help:
      | An explicitly laid-out delay line to avoid mapping to SRL16s
      | for use in pipelining to help achieve timing closure.
      mask init:
      | pipeline_init(gcb,'latency',csp_latency);
      settings: AttributesFormatString=Latency = %<latency>
      mask Display:
      | port_label('input', 1, 'd');
      | port_label('output', 1, 'q');
      | disp(['Z^-', num2str(csp_latency)]);
  pipeline44 : Subsystem  Tag=cmac_delinked  mask(pipeline){csp_latency=2}
      mask prompts: csp_latency "Latency"
      mask help:
      | An explicitly laid-out delay line to avoid mapping to SRL16s
      | for use in pipelining to help achieve timing closure.
      mask init:
      | pipeline_init(gcb,'latency',csp_latency);
      settings: AttributesFormatString=Latency = %<latency>
      mask Display:
      | port_label('input', 1, 'd');
      | port_label('output', 1, 'q');
      | disp(['Z^-', num2str(csp_latency)]);
  pipeline48 : Subsystem  Tag=cmac_delinked  mask(pipeline){csp_latency=2}
      mask prompts: csp_latency "Latency"
      mask help:
      | An explicitly laid-out delay line to avoid mapping to SRL16s
      | for use in pipelining to help achieve timing closure.
      mask init:
      | pipeline_init(gcb,'latency',csp_latency);
      settings: AttributesFormatString=Latency = %<latency>
      mask Display:
      | port_label('input', 1, 'd');
      | port_label('output', 1, 'q');
      | disp(['Z^-', num2str(csp_latency)]);
  pipeline5 : Subsystem  Tag=cmac_delinked  mask(pipeline){csp_latency=2}
      mask prompts: csp_latency "Latency"
      mask help:
      | An explicitly laid-out delay line to avoid mapping to SRL16s
      | for use in pipelining to help achieve timing closure.
      mask init:
      | pipeline_init(gcb,'latency',csp_latency);
      settings: AttributesFormatString=Latency = %<latency>
      mask Display:
      | port_label('input', 1, 'd');
      | port_label('output', 1, 'q');
      | disp(['Z^-', num2str(csp_latency)]);
  pipeline50 : Subsystem  Tag=cmac_delinked  mask(pipeline){csp_latency=2}
      mask prompts: csp_latency "Latency"
      mask help:
      | An explicitly laid-out delay line to avoid mapping to SRL16s
      | for use in pipelining to help achieve timing closure.
      mask init:
      | pipeline_init(gcb,'latency',csp_latency);
      settings: AttributesFormatString=Latency = %<latency>
      mask Display:
      | port_label('input', 1, 'd');
      | port_label('output', 1, 'q');
      | disp(['Z^-', num2str(csp_latency)]);
  pipeline6 : Subsystem  Tag=cmac_delinked  mask(pipeline){csp_latency=2}
      mask prompts: csp_latency "Latency"
      mask help:
      | An explicitly laid-out delay line to avoid mapping to SRL16s
      | for use in pipelining to help achieve timing closure.
      mask init:
      | pipeline_init(gcb,'latency',csp_latency);
      settings: AttributesFormatString=Latency = %<latency>
      mask Display:
      | port_label('input', 1, 'd');
      | port_label('output', 1, 'q');
      | disp(['Z^-', num2str(csp_latency)]);
  pipeline7 : Subsystem  Tag=cmac_delinked  mask(pipeline){csp_latency=2}
      mask prompts: csp_latency "Latency"
      mask help:
      | An explicitly laid-out delay line to avoid mapping to SRL16s
      | for use in pipelining to help achieve timing closure.
      mask init:
      | pipeline_init(gcb,'latency',csp_latency);
      settings: AttributesFormatString=Latency = %<latency>
      mask Display:
      | port_label('input', 1, 'd');
      | port_label('output', 1, 'q');
      | disp(['Z^-', num2str(csp_latency)]);
  pipeline8 : Subsystem  Tag=cmac_delinked  mask(pipeline){csp_latency=2}
      mask prompts: csp_latency "Latency"
      mask help:
      | An explicitly laid-out delay line to avoid mapping to SRL16s
      | for use in pipelining to help achieve timing closure.
      mask init:
      | pipeline_init(gcb,'latency',csp_latency);
      settings: AttributesFormatString=Latency = %<latency>
      mask Display:
      | port_label('input', 1, 'd');
      | port_label('output', 1, 'q');
      | disp(['Z^-', num2str(csp_latency)]);
  pipeline9 : Subsystem  Tag=cmac_delinked  mask(pipeline){csp_latency=2}
      mask prompts: csp_latency "Latency"
      mask help:
      | An explicitly laid-out delay line to avoid mapping to SRL16s
      | for use in pipelining to help achieve timing closure.
      mask init:
      | pipeline_init(gcb,'latency',csp_latency);
      settings: AttributesFormatString=Latency = %<latency>
      mask Display:
      | port_label('input', 1, 'd');
      | port_label('output', 1, 'q');
      | disp(['Z^-', num2str(csp_latency)]);
  pulse_ext : Subsystem  mask(pulse_ext){pulse_len=10}
      mask prompts: pulse_len "Length of Pulse"
      mask help:
      | Extends a boolean signal to be high for the specified number of clocks after
      | the last high input.
      mask init:
      | bits = ceil(log2(pulse_len+1));
      mask Help: eval('xlWeb(''http://casper.berkeley.edu/wiki/Pulse_ext'')')
  pulse_ext1 : Subsystem  mask(pulse_ext){pulse_len=10}
      mask prompts: pulse_len "Length of Pulse"
      mask help:
      | Extends a boolean signal to be high for the specified number of clocks after
      | the last high input.
      mask init:
      | bits = ceil(log2(pulse_len+1));
      mask Help: eval('xlWeb(''http://casper.berkeley.edu/wiki/Pulse_ext'')')
  pulse_ext2 : Subsystem  mask(pulse_ext){pulse_len=10}
      mask prompts: pulse_len "Length of Pulse"
      mask help:
      | Extends a boolean signal to be high for the specified number of clocks after
      | the last high input.
      mask init:
      | bits = ceil(log2(pulse_len+1));
      mask Help: eval('xlWeb(''http://casper.berkeley.edu/wiki/Pulse_ext'')')
  pulse_ext3 : Subsystem  mask(pulse_ext){pulse_len=10}
      mask prompts: pulse_len "Length of Pulse"
      mask help:
      | Extends a boolean signal to be high for the specified number of clocks after
      | the last high input.
      mask init:
      | bits = ceil(log2(pulse_len+1));
      mask Help: eval('xlWeb(''http://casper.berkeley.edu/wiki/Pulse_ext'')')
  snap_fft : Subsystem  Tag=casper:bitsnap  AncestorBlock=casper_library_scopes/bitfield_snapshot  mask(bitsnap){io_names=[fft_re fft_im ch of dv sync cnt_sync], io_widths=[22 22 15 1 1 1 1], io_bps=[21 21 0 0 0 0 0], io_types=[1 1 0 2 2 2 2], show_format=on, snap_storage=bram, snap_dram_dimm=2, snap_dram_clock=250, snap_nsamples=13, snap_data_width=64, snap_offset=on, snap_circap=off, snap_value=off, snap_ext_arm=off, snap_ext_circ=off, snap_provide_outputs=on, snap_use_dsp48=on, snap_delay=0, extra_names=[c d], extra_widths=[30 2], extra_bps=[0 0], extra_types=0}
      mask prompts: io_names "Names [msb...lsb]"; io_widths "Bitwidths [msb...lsb]"; io_bps "Binary pts [msb...lsb]"; io_types "Data types [msb...lsb], ufix=0, fix=1, bool=2"; show_format "Print format string?"; snap_storage "Storage medium"; snap_dram_dimm "DRAM dimm"; snap_dram_clock "DRAM clock rate"; snap_nsamples "Number of Samples (2^?)"; snap_data_width "Data width"; snap_offset "Start delay support"; snap_circap "Circular capture support"; snap_value "Extra value capture support"; snap_ext_arm "External arm support"; snap_ext_circ "External circular capture support"; snap_provide_outputs "Provide outputs"; snap_use_dsp48 "Use DSP48s to implement counters"; snap_delay "Pre-snapshot delay"; extra_names "Names [msb...lsb]"; extra_widths "Widths [msb...lsb]"; extra_bps "Binary pts [msb...lsb]"; extra_types "Data types [msb...lsb], ufix=0, fix=1, bool=2"
      mask help:
      | A wrapped snapshot block. Allows specification of inputs to a snapblock word so the toolflow can automatically set up the scope.
      | See documentation for snapshot for explanation of parameters.
      mask init:
      | bitsnap_init(gcb);
      settings: AttributesFormatString=|
      | snap(7):f22.21,f22.21,uf15.0,b,b,b,b = 63 bits\n64 wide, 8192 deep
      | debugID: 113542023
      mask TypeOptions snap_storage: bram | dram
      mask Callback snap_storage: bitsnap_callback();
      mask TypeOptions snap_dram_dimm: 1 | 2 | 3 | 4
      mask TypeOptions snap_dram_clock: 200 | 250 | 266 | 300 | 333
      mask TypeOptions snap_data_width: 8 | 16 | 32 | 64 | 128
      mask Callback snap_value: bitsnap_callback();
      mask Callback snap_ext_arm: bitsnap_callback();
      mask Callback snap_ext_circ: bitsnap_callback();
      mask Callback snap_provide_outputs: bitsnap_callback();
      mask DialogControl ParameterTabVar0 Prompt: Inputs
      mask DialogControl ParameterTabVar01 Prompt: Snapshot
      mask DialogControl ParameterTabVar012 Prompt: Extra Value
  sync_gen : Subsystem
  sync_out : Outport
  dv_out : Outport  Port=2
  pol0_out : Outport  Port=3
  pol1_out : Outport  Port=4
  pfb_of : Outport  Port=5
  pfb_ch_out : Outport  Port=6
  tag scope: current_channel=global, data_pol0=global, fft_ch0=global, fft_ch1=global, fft_dv0=global, fft_dv1=global, fft_dvalid=global, fft_p0_fifo_full=global, fft_p1_fifo_full=global, fft_pol0_err=global, fft_pol0_of=global, fft_pol1_err=global, fft_pol1_of=global, fft_sync0=global, fft_sync=global, fft_tready_p0=global, fft_tready_p1=global, fir_data_tlast=global, fir_dvalid_pol0=global, fir_pol0=global, fir_sync=global, reg_channel=global, reord_channel=global, reord_dv=global, reord_mux_sel=global, reord_mux_sel_ext=global, reord_pol0=global, reord_pol1=global, reord_sync=global
  wires:
  pol0/1 -> bus_scale2/1(din)
  pol1/1 -> bus_scale1/1(din)
  sync/1 -> Terminator5/1, Delay/1
  Reinterpret2/1 -> Concat3/1
  Reinterpret3/1 -> Concat3/2
  Concat3/1 -> [data_pol1]
  Gateway Out6/1 -> To Workspace6/1
  Gateway Out1/1 -> To Workspace1/1
  Gateway Out36/1 -> To Workspace36/1
  [fft_im_pol1] -> Reinterpret3/1
  [fft_re_pol1] -> Reinterpret2/1
  dvalid/1 -> Gateway Out36/1, Delay22/1, Delay20/1
  Counter3/1 -> Relational4/1, Gateway Out53/1
  Constant9/1 -> Relational4/2
  Gateway Out70/1 -> To Workspace69/1
  Gateway Out71/1 -> To Workspace70/1
  From28/1 -> Gateway Out70/1
  From33/1 -> Gateway Out71/1
  fft_shift/1 -> [fft_shift]
  pipeline19/1(q) -> [fir_dvalid_pol0], Gateway Out1/1, Counter3/2
  "Fast Fourier Transform 9.1 "/2 -> [fft_tready_p0], Inverter5/1
  pipeline110/1(q) -> [fft_ch0]
  Gateway Out66/1 -> To Workspace65/1
  Gateway Out67/1 -> To Workspace66/1
  From40/1 -> Gateway Out67/1
  From38/1 -> Gateway Out66/1
  "Fast Fourier Transform 9.1 "/5 -> pipeline122/1(d)
  "Fast Fourier Transform 9.1 "/6 -> pipeline123/1(d)
  "Fast Fourier Transform 9.1 "/8 -> sync_gen/1(In1), pipeline110/1(d)
  "Fast Fourier Transform 9.1 "/15 -> Terminator7/1
  "Fast Fourier Transform 9.1 "/16 -> Terminator8/1
  "Fast Fourier Transform 9.1 "/17 -> Terminator9/1
  pipeline123/1(q) -> [fft_re_pol0_int]
  pipeline122/1(q) -> [fft_im_pol0_int]
  Inverter1/1 -> "Fast Fourier Transform 9.1 "/10, Logical9/2
  Gateway Out37/1 -> To Workspace37/1
  [fir_sync] -> pulse_ext/1(in), Delay9/1
  From108/1 -> Gateway Out37/1
  Concat/1 -> [data_pol0]
  Gateway Out34/1 -> To Workspace32/1
  [fft_sync0] -> [fft_sync]
  From2/1 -> Gateway Out34/1
  [fft_ch0] -> [current_channel]
  [fft_im_pol0] -> Reinterpret1/1
  [fft_re_pol0] -> Reinterpret/1
  From140/1 -> bus_expand16/1(bus_in)
  Gateway Out2/1 -> To Workspace2/1
  Gateway Out5/1 -> To Workspace5/1
  [fft_dv0] -> [fft_dvalid]
  From26/1 -> pipeline27/1(d)
  Counter4/1 -> Goto29/1, fft_sync_cnt/1(out_reg)
  pipeline1/1(q) -> Counter4/2
  pipeline27/1(q) -> Counter4/1
  From32/1 -> pipeline1/1(d)
  Gateway Out18/1 -> To Workspace19/1
  Gateway Out7/1 -> To Workspace7/1
  Gateway Out83/1 -> To Workspace85/1
  [sync_out] -> Gateway Out7/1, sync_out/1
  [pol0] -> pol0_out/1
  [pol1] -> pol1_out/1
  [nb_dv] -> Gateway Out18/1, dv_out/1
  Constant12/1 -> "Fast Fourier Transform 9.1 "/8
  Constant10/1 -> "Fast Fourier Transform 9.1 "/3
  Constant3/1 -> "Fast Fourier Transform 9.1 "/2
  Constant13/1 -> Fast Fourier Transform 9.1 1/3
  bus_expand1/2(lsb_out1) -> Fast Fourier Transform 9.1 1/4
  bus_expand1/1(msb_out2) -> Fast Fourier Transform 9.1 1/5
  [fir_data_tlast] -> Fast Fourier Transform 9.1 1/7
  Constant8/1 -> Fast Fourier Transform 9.1 1/9
  pipeline124/1(q) -> [fft_dv0]
  From4/1 -> bus_expand13/1(bus_in)
  Gateway Out4/1 -> To Workspace4/1
  bus_expand13/1(msb_out2) -> Gateway Out4/1
  Gateway Out8/1 -> To Workspace8/1
  bus_expand13/2(lsb_out1) -> Gateway Out8/1
  [data_pol0] -> Delay88/1, Delay46/1
  Delay24/1 -> Delay4/1
  [fft_sync] -> Register12/3, Register12/1
  Gateway Out15/1 -> To Workspace15/1
  Gateway Out17/1 -> To Workspace17/1
  [current_channel] -> Slice2/1, Slice4/1
  Constant17/1 -> AddSub/2
  AddSub/1 -> Delay3/1
  Delay12/1 -> Single Port RAM/2
  Delay18/1 -> Single Port RAM/1
  Delay46/1 -> Delay12/1
  Delay47/1 -> Delay18/1
  Delay3/1 -> Delay99/1
  Reinterpret1/1 -> Concat/2
  Reinterpret/1 -> Concat/1
  bus_expand3/2(lsb_out1) -> Gateway Out17/1
  bus_expand3/1(msb_out2) -> Gateway Out15/1
  Gateway Out50/1 -> To Workspace51/1
  Gateway Out51/1 -> To Workspace3/1
  Gateway Out52/1 -> To Workspace16/1
  bus_expand16/1(msb_out2) -> Gateway Out2/1
  bus_expand16/2(lsb_out1) -> Gateway Out5/1
  From30/1 -> Gateway Out51/1
  From20/1 -> Gateway Out52/1
  Gateway Out3/1 -> To Workspace47/1
  Delay55/1 -> Delay49/1
  Gateway Out16/1 -> To Workspace42/1
  From123/1 -> bus_expand3/1(bus_in)
  From124/1 -> Gateway Out50/1
  Delay48/1 -> Delay21/1
  From125/1 -> Gateway Out3/1
  From126/1 -> Gateway Out16/1
  Logical6/1 -> Delay24/1
  [fft_dvalid] -> Logical6/1
  Inverter/1 -> Logical6/2
  Mux1/1 -> [reord_pol0]
  Single Port RAM/1 -> Mux1/2
  Delay92/1 -> Delay45/1, AddSub/1
  [current_channel] -> Delay92/1
  Delay88/1 -> Delay93/1
  Delay93/1 -> Delay94/1
  Delay94/1 -> Mux1/3
  Delay113/1 -> Mux1/1, Delay114/1
  Delay4/1 -> Single Port RAM/3
  Slice4/1 -> Delay47/1
  Logical8/1 -> Register12/2, Delay55/1
  Register12/1 -> Logical8/2
  [fft_dvalid] -> Logical5/1, Delay95/1
  Delay50/1 -> Delay48/1
  Delay95/1 -> Delay50/1
  [data_pol1] -> Delay91/1, Delay101/1
  [current_channel] -> Slice6/1, Slice3/1
  Slice3/1 -> Delay115/1, Inverter3/1
  Delay65/1 -> Single Port RAM1/1
  Delay87/1 -> Delay90/1
  Delay91/1 -> Delay63/1
  Delay96/1 -> Delay65/1
  Logical10/1 -> Delay87/1
  [fft_dvalid] -> Logical10/1
  Inverter3/1 -> Logical10/2
  Single Port RAM1/1 -> Mux11/2
  Delay101/1 -> Delay103/1
  Delay103/1 -> Delay104/1
  Delay104/1 -> Mux11/3
  Delay117/1 -> Mux11/1
  Delay90/1 -> Single Port RAM1/3
  Slice6/1 -> Delay96/1
  Mux11/1 -> [reord_pol1]
  Gateway Out48/1 -> To Workspace53/1
  Gateway Out53/1 -> To Workspace54/1
  Relational4/1 -> Gateway Out48/1, [fir_data_tlast]
  Delay21/1 -> [reord_dv]
  Delay99/1 -> [reord_channel]
  Delay63/1 -> Single Port RAM1/2
  Logical5/1 -> Delay102/1
  Slice2/1 -> Delay111/1, [reord_mux_sel], Inverter/1
  [reord_mux_sel] -> Logical5/2
  Delay45/1 -> Delay86/1
  Delay86/1 -> Delay100/1
  Gateway Out57/1 -> To Workspace58/1
  Delay100/1 -> Gateway Out57/1, [reg_channel]
  Delay102/1 -> Logical8/1
  Delay49/1 -> Delay110/1
  pipeline17/1(q) -> [fir_sync], Gateway Out6/1, Counter3/1
  Delay110/1 -> [reord_sync]
  [fft_ch_out] -> pfb_ch_out/1, Gateway Out83/1
  Delay111/1 -> Delay112/1
  Delay112/1 -> Delay113/1
  Delay114/1 -> [reord_mux_sel_ext]
  Delay116/1 -> Delay117/1
  Delay115/1 -> Delay116/1
  Fast Fourier Transform 9.1 1/1 -> Terminator1/1
  Fast Fourier Transform 9.1 1/10 -> Terminator12/1
  Fast Fourier Transform 9.1 1/17 -> Terminator4/1
  Fast Fourier Transform 9.1 1/16 -> Terminator3/1
  Fast Fourier Transform 9.1 1/15 -> Terminator2/1
  Fast Fourier Transform 9.1 1/13 -> Terminator11/1
  Fast Fourier Transform 9.1 1/11 -> Terminator13/1
  Fast Fourier Transform 9.1 1/12 -> Terminator21/1
  Fast Fourier Transform 9.1 1/2 -> Inverter8/1, [fft_tready_p1]
  Constant5/1 -> Fast Fourier Transform 9.1 1/2
  Fast Fourier Transform 9.1 1/3 -> Terminator15/1
  Fast Fourier Transform 9.1 1/4 -> Terminator16/1
  [fft_pol1_of] -> Concat2/2
  [fft_pol0_of] -> Concat2/1
  Concat2/1 -> pfb_of/1
  Constant4/1 -> "Fast Fourier Transform 9.1 "/9
  Constant11/1 -> Fast Fourier Transform 9.1 1/8
  "Fast Fourier Transform 9.1 "/3 -> Terminator17/1
  "Fast Fourier Transform 9.1 "/4 -> Terminator18/1
  "Fast Fourier Transform 9.1 "/13 -> Terminator20/1
  "Fast Fourier Transform 9.1 "/12 -> Terminator22/1
  "Fast Fourier Transform 9.1 "/11 -> Terminator23/1
  "Fast Fourier Transform 9.1 "/10 -> Terminator24/1
  pipeline16/1(q) -> [fft_pol0_of]
  "Fast Fourier Transform 9.1 "/7 -> Terminator19/1
  "Fast Fourier Transform 9.1 "/14 -> pipeline16/1(d)
  Fast Fourier Transform 9.1 1/14 -> pipeline5/1(d)
  Fast Fourier Transform 9.1 1/7 -> Terminator10/1
  pipeline50/1(q) -> [fft_dv1]
  [fft_shift] -> "Fast Fourier Transform 9.1 "/1
  "Fast Fourier Transform 9.1 "/9 -> Logical9/1
  Logical9/1 -> sync_gen/2(In2), pipeline124/1(d)
  bus_expand2/1(msb_out2) -> "Fast Fourier Transform 9.1 "/5
  bus_expand2/2(lsb_out1) -> "Fast Fourier Transform 9.1 "/4
  [fir_data_tlast] -> "Fast Fourier Transform 9.1 "/7
  Logical12/1 -> [fft_pol0_err]
  Inverter5/1 -> Logical12/1
  pulse_ext/1(out) -> Inverter1/1
  [fir_dvalid_pol0] -> Delay2/1
  FIFO/3 -> [fft_p0_fifo_full]
  FIFO/2 -> Inverter6/1
  [fir_pol0] -> Delay6/1
  pulse_ext1/1(out) -> Inverter7/1, FIFO/4
  Logical1/1 -> FIFO/2
  Inverter7/1 -> Logical1/2
  [fir_sync] -> pulse_ext1/1(in)
  Delay2/1 -> Logical1/1
  Delay6/1 -> FIFO/1
  Logical13/1 -> "Fast Fourier Transform 9.1 "/6, Logical12/2
  [fft_tready_p0] -> Logical13/2, FIFO/3
  Inverter6/1 -> Logical13/1
  pipeline21/1(q) -> [fir_dvalid_pol1]
  pulse_ext2/1(out) -> Inverter2/1
  Inverter2/1 -> Logical7/2, Fast Fourier Transform 9.1 1/10
  [fir_sync] -> pulse_ext2/1(in)
  Fast Fourier Transform 9.1 1/9 -> Logical7/1
  Logical7/1 -> pipeline50/1(d)
  Fast Fourier Transform 9.1 1/5 -> pipeline44/1(d)
  Fast Fourier Transform 9.1 1/6 -> pipeline48/1(d)
  pipeline44/1(q) -> [fft_im_pol1_int]
  pipeline48/1(q) -> [fft_re_pol1_int]
  Fast Fourier Transform 9.1 1/8 -> pipeline12/1(d)
  Inverter8/1 -> Logical11/1
  Logical14/1 -> Fast Fourier Transform 9.1 1/6, Logical11/2
  [fft_shift] -> Fast Fourier Transform 9.1 1/1
  FIFO1/2 -> Inverter9/1
  pulse_ext3/1(out) -> Inverter10/1, FIFO1/4
  Logical2/1 -> FIFO1/2
  Inverter10/1 -> Logical2/2
  Delay8/1 -> Logical2/1
  Delay11/1 -> FIFO1/1
  [fft_tready_p1] -> Logical14/2, FIFO1/3
  Inverter9/1 -> Logical14/1
  [fir_dvalid_pol1] -> Delay8/1
  [fir_pol1] -> Delay11/1
  [fir_sync] -> pulse_ext3/1(in)
  "Fast Fourier Transform 9.1 "/1 -> Terminator6/1
  [fft_im_pol0_int] -> [fft_im_pol0]
  [fft_re_pol0_int] -> [fft_re_pol0]
  [reord_sync] -> [sync_out]
  [reord_dv] -> Delay5/1
  [reord_pol0] -> Delay7/1
  [reord_pol1] -> Delay10/1
  Delay9/1 -> sync_gen/3(In3)
  sync_gen/1(Out1) -> [fft_sync0]
  [reord_channel] -> Delay1/1
  From31/1 -> Logical4/1
  From34/1 -> Logical4/2
  Counter5/1 -> fft_sync_align/1(out_reg)
  Logical4/1 -> Counter5/2
  From42/1 -> Counter5/1
  FIFO1/3 -> [fft_p1_fifo_full]
  [fft_re_pol1_int] -> [fft_re_pol1]
  [fft_im_pol1_int] -> [fft_im_pol1]
  pipeline12/1(q) -> [fft_ch1]
  pipeline5/1(q) -> [fft_pol1_of]
  Logical11/1 -> [fft_pol1_err]
  Delay1/1 -> [fft_ch_out]
  Delay5/1 -> [nb_dv]
  Delay7/1 -> [pol0]
  Delay10/1 -> [pol1]
  FIFO/1 -> bus_convert/1(din)
  FIFO1/1 -> bus_convert1/1(din)
  bus_convert/1(dout) -> bus_expand2/1(bus_in)
  bus_convert1/1(dout) -> bus_expand1/1(bus_in)
  [nb_dv] -> pipeline7/1(d)
  [fft_pol0_of] -> pipeline6/1(d)
  bus_expand4/2(lsb_out1) -> pipeline3/1(d)
  [pol0] -> bus_expand4/1(bus_in)
  bus_expand4/1(msb_out2) -> pipeline2/1(d)
  pipeline2/1(q) -> Delay19/1
  pipeline3/1(q) -> Delay17/1
  pipeline4/1(q) -> Delay16/1
  pipeline6/1(q) -> Delay15/1
  pipeline7/1(q) -> Delay14/1
  [fft_ch_out] -> Relational/1, pipeline4/1(d)
  pipeline8/1(q) -> Delay13/1
  pipeline10/1(q) -> Relational/2
  Constant1/1 -> fft_trig_thresh/1(sim_1)
  fft_trig_thresh/1(in_threshold) -> pipeline10/1(d)
  edge_detect65/1(out) -> snap_fft/7(in_cnt_sync), snap_fft/9(trig)
  [sync_out] -> Mux/2, pipeline8/1(d)
  Relational/1 -> Mux/3
  Mux/1 -> edge_detect65/1(in)
  fft_trig_sel/1(in_sel) -> pipeline9/1(d)
  Constant2/1 -> fft_trig_sel/1(sim_1)
  pipeline9/1(q) -> Mux/1
  Delay13/1 -> snap_fft/6(in_sync)
  Delay14/1 -> snap_fft/8(we), snap_fft/5(in_dv)
  Delay15/1 -> snap_fft/4(in_of)
  Delay16/1 -> snap_fft/3(in_ch)
  Delay17/1 -> snap_fft/2(in_fft_im)
  Delay19/1 -> snap_fft/1(in_fft_re)
  pipeline18/1(q) -> [fir_pol0]
  pipeline20/1(q) -> [fir_pol1]
  bus_scale2/1(dout) -> bus_convert2/1(din)
  bus_scale1/1(dout) -> bus_convert3/1(din)
  bus_convert2/1(dout) -> pipeline18/1(d)
  bus_convert3/1(dout) -> pipeline20/1(d)
  Delay/1 -> pipeline17/1(d)
  Delay20/1 -> pipeline19/1(d)
  Delay22/1 -> pipeline21/1(d)
